simulink model "Robot2R_dyn"  (R2025b)
settings: Solver=VariableStepAuto  StartTime=0.0  StopTime=10.0  RelTol=1e-3  AbsTol=1e-3
undefined symbols (not defined in the file): X, Y, Z
libraries: sm_lib x20, nesl_utility x19, robotcorelib x2, simulink x1
settings Model: Creator=samu0  LastModifiedBy=samuisa
settings SolverCC: AutoScaleAbsTol=off  AlgebraicLoopSolver=TrustRegion  MaxZcPerStep=1.0
settings DebuggingCC: UnconnectedInputMsg=warning  UnconnectedOutputMsg=warning  UnconnectedLineMsg=warning  SymbolicDimsDataTypeCodeGenerationDiagnostic=none
settings ModelReferenceCC: EnableRefExpFcnMdlSchedulingChecks=on
settings SFSimCC: CustomCodeUndefinedFunction=UseInterfaceOnly
settings RTWCC: GPUComputeCapability=3.5  DLArmComputeVersion=19.05
settings SimscapeCC: SimscapeLogType=all  SimscapeLogSimulationStatistics=on  SimscapeLogDataHistory=10000.0

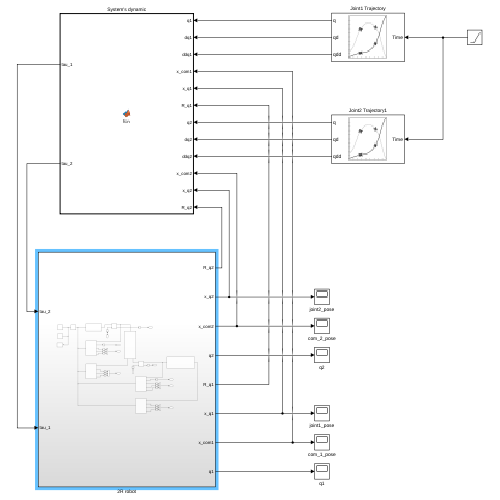
[thumbnail: Simulink's stored preview of the top-level diagram]
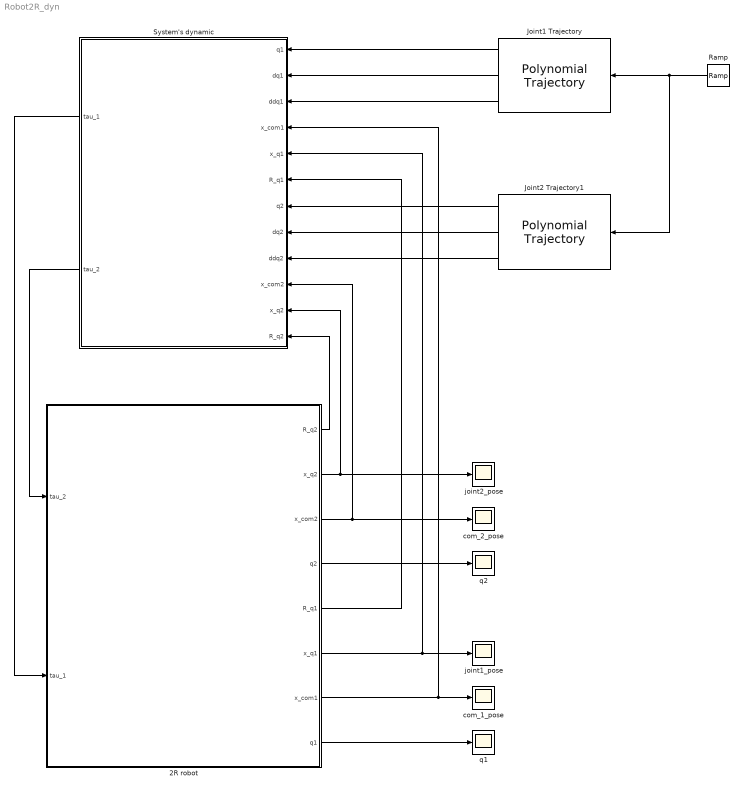
== system Robot2R_dyn ==
  2R robot : Subsystem
  Joint1 Trajectory : robotcorelib/Polynomial Trajectory  WaypointSource=Internal  Waypoints=[ 0, 1.57/2 ]  TimePoints=[ 0, 20 ]  TimeInterval=[ 1, 4 ]  Method=Cubic Polynomial  ParameterSource=Internal  VelocityBoundaryCondition=zeros( 1,2 )  AccelerationBoundaryCondition=zeros( 2, 5 )  SimulateUsing=Interpreted execution
  Joint2 Trajectory1 : robotcorelib/Polynomial Trajectory  WaypointSource=Internal  Waypoints=[ 0, 0 ]  TimePoints=[ 0, 20 ]  TimeInterval=[ 1, 4 ]  Method=Cubic Polynomial  ParameterSource=Internal  VelocityBoundaryCondition=zeros( 1,2 )  AccelerationBoundaryCondition=zeros( 2, 5 )  SimulateUsing=Interpreted execution
  Ramp : simulink/Sources/Ramp  slope=1  start=0  InitialOutput=0
  System's dynamic : MATLAB Function  TreatAsAtomicUnit=on
  com_1_pose : Scope
      settings: ActiveDisplayYMinimum=-1  ActiveDisplayYMaximum=1  DataLoggingVariableName=ScopeData3
  com_2_pose : Scope
      settings: DataLoggingVariableName=ScopeData5
  joint1_pose : Scope
      settings: ActiveDisplayYMinimum=-1  ActiveDisplayYMaximum=1  DataLoggingVariableName=ScopeData2
  joint2_pose : Scope
      settings: DataLoggingVariableName=ScopeData4
  q1 : Scope
  q2 : Scope
  wires:
  System's dynamic/2(tau_2) -> 2R robot/1(tau_2)
  2R robot/7(x_com1) -> com_1_pose/1, System's dynamic/4(x_com1)
  2R robot/3(x_com2) -> com_2_pose/1, System's dynamic/10(x_com2)
  2R robot/8(q1) -> q1/1
  2R robot/4(q2) -> q2/1
  2R robot/2(x_q2) -> joint2_pose/1, System's dynamic/11(x_q2)
  2R robot/6(x_q1) -> joint1_pose/1, System's dynamic/5(x_q1)
  System's dynamic/1(tau_1) -> 2R robot/2(tau_1)
  2R robot/5(R_q1) -> System's dynamic/6(R_q1)
  2R robot/1(R_q2) -> System's dynamic/12(R_q2)
  Joint1 Trajectory/1 -> System's dynamic/1(q1)
  Joint1 Trajectory/2 -> System's dynamic/2(dq1)
  Joint1 Trajectory/3 -> System's dynamic/3(ddq1)
  Joint2 Trajectory1/1 -> System's dynamic/7(q2)
  Joint2 Trajectory1/2 -> System's dynamic/8(dq2)
  Joint2 Trajectory1/3 -> System's dynamic/9(ddq2)
  Ramp/1 -> Joint2 Trajectory1/1, Joint1 Trajectory/1

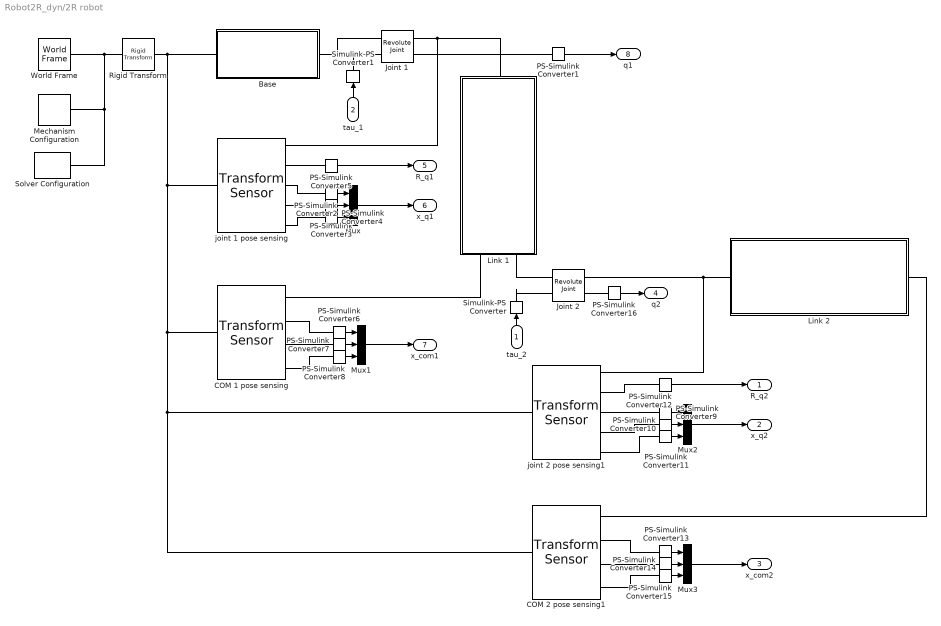
== system Robot2R_dyn/2R robot ==
  tau_2 : Inport
  tau_1 : Inport  Port=2
  Base : Subsystem
  COM 1 pose sensing : sm_lib/Frames and Transforms/Transform Sensor  MeasurementFrame=Base  RotationSequence=XYX  SenseAngle=off  SenseAxis=off  SenseQ=off  SenseR=off  SenseRotationSequence=off  SenseOmegaX=off  SenseOmegaY=off  SenseOmegaZ=off  SenseOmega=off  SenseQDot=off  SenseRDot=off  SenseRotationSequenceDot=off  SenseAlphaX=off  SenseAlphaY=off  SenseAlphaZ=off  SenseAlpha=off  SenseQDDot=off  SenseRDDot=off  SenseX=on  SenseY=on  SenseZ=on  SenseXYZ=off  SenseRad=off  SenseAzim=off  SenseDist=off  SenseInc=off  SenseXDot=off  SenseYDot=off  SenseZDot=off  SenseXYZDot=off  SenseRadDot=off  SenseAzimDot=off  SenseDistDot=off  SenseIncDot=off  SenseXDDot=off  SenseYDDot=off  SenseZDDot=off  SenseXYZDDot=off  SenseRadDDot=off  SenseAzimDDot=off  SenseDistDDot=off  SenseIncDDot=off
  COM 2 pose sensing1 : sm_lib/Frames and Transforms/Transform Sensor  MeasurementFrame=Base  RotationSequence=XYX  SenseAngle=off  SenseAxis=off  SenseQ=off  SenseR=off  SenseRotationSequence=off  SenseOmegaX=off  SenseOmegaY=off  SenseOmegaZ=off  SenseOmega=off  SenseQDot=off  SenseRDot=off  SenseRotationSequenceDot=off  SenseAlphaX=off  SenseAlphaY=off  SenseAlphaZ=off  SenseAlpha=off  SenseQDDot=off  SenseRDDot=off  SenseX=on  SenseY=on  SenseZ=on  SenseXYZ=off  SenseRad=off  SenseAzim=off  SenseDist=off  SenseInc=off  SenseXDot=off  SenseYDot=off  SenseZDot=off  SenseXYZDot=off  SenseRadDot=off  SenseAzimDot=off  SenseDistDot=off  SenseIncDot=off  SenseXDDot=off  SenseYDDot=off  SenseZDDot=off  SenseXYZDDot=off  SenseRadDDot=off  SenseAzimDDot=off  SenseDistDDot=off  SenseIncDDot=off
  Joint 1 : sm_lib/Joints/Revolute Joint  JointMode=Normal  CompositeWrenchDir=FollowerOnBase  CompositeWrenchFrame=BaseFrame  SenseConstraintForce=off  SenseConstraintTorque=off  SenseTotalForce=off  SenseTotalTorque=off  PositionTargetSpecify=off  PositionTargetPriority=High  PositionTargetValue=0  PositionTargetValueUnits=deg  VelocityTargetSpecify=off  VelocityTargetPriority=High  VelocityTargetValue=0  VelocityTargetValueUnits=deg/s  EquilibriumPosition=0  EquilibriumPositionUnits=rad  SpringStiffness=0  SpringStiffnessUnits=N*m/rad  DampingCoefficient=0.002  DampingCoefficientUnits=N*m*s/rad  LowerLimitSpecify=off  LowerLimitBound=-90  LowerLimitBoundUnits=deg  LowerLimitStiffness=1e4  LowerLimitStiffnessUnits=N*m/deg  LowerLimitDamping=10  LowerLimitDampingUnits=N*m/(deg/s)  LowerLimitTransitionRegionWidth=0.1  LowerLimitTransitionRegionWidthUnits=deg  UpperLimitSpecify=off  UpperLimitBound=90  UpperLimitBoundUnits=deg  UpperLimitStiffness=1e4  UpperLimitStiffnessUnits=N*m/deg  UpperLimitDamping=10  UpperLimitDampingUnits=N*m/(deg/s)  UpperLimitTransitionRegionWidth=0.1  UpperLimitTransitionRegionWidthUnits=deg  TorqueActuationMode=InputTorque  MotionActuationMode=ComputedMotion  SensePosition=on  SenseVelocity=off  SenseAcceleration=off  SenseTorqueForce=off  SenseLowerLimitTorqueForce=off  SenseUpperLimitTorqueForce=off
  Joint 2 : sm_lib/Joints/Revolute Joint  JointMode=Normal  CompositeWrenchDir=FollowerOnBase  CompositeWrenchFrame=BaseFrame  SenseConstraintForce=off  SenseConstraintTorque=off  SenseTotalForce=off  SenseTotalTorque=off  PositionTargetSpecify=off  PositionTargetPriority=High  PositionTargetValue=0  PositionTargetValueUnits=deg  VelocityTargetSpecify=off  VelocityTargetPriority=High  VelocityTargetValue=0  VelocityTargetValueUnits=deg/s  EquilibriumPosition=0  EquilibriumPositionUnits=rad  SpringStiffness=0  SpringStiffnessUnits=N*m/rad  DampingCoefficient=0.002  DampingCoefficientUnits=N*m*s/rad  LowerLimitSpecify=off  LowerLimitBound=-90  LowerLimitBoundUnits=deg  LowerLimitStiffness=1e4  LowerLimitStiffnessUnits=N*m/deg  LowerLimitDamping=10  LowerLimitDampingUnits=N*m/(deg/s)  LowerLimitTransitionRegionWidth=0.1  LowerLimitTransitionRegionWidthUnits=deg  UpperLimitSpecify=off  UpperLimitBound=90  UpperLimitBoundUnits=deg  UpperLimitStiffness=1e4  UpperLimitStiffnessUnits=N*m/deg  UpperLimitDamping=10  UpperLimitDampingUnits=N*m/(deg/s)  UpperLimitTransitionRegionWidth=0.1  UpperLimitTransitionRegionWidthUnits=deg  TorqueActuationMode=InputTorque  MotionActuationMode=ComputedMotion  SensePosition=on  SenseVelocity=off  SenseAcceleration=off  SenseTorqueForce=off  SenseLowerLimitTorqueForce=off  SenseUpperLimitTorqueForce=off
  Link 1 : Subsystem
  Link 2 : Subsystem
  Mechanism Configuration : sm_lib/Utilities/Mechanism Configuration  UniformGravity=Constant  GravityVector=[0 0 -9.81]  GravityVectorUnits=m/s^2  LinearizationDelta=0.001  JointModeTransitionNonlinearIterations=2
  Mux{,1..3} (4 alike) : Mux  Inputs=3
  PS-Simulink Converter{1..16} (16 alike) : nesl_utility/PS-Simulink Converter  PhysicalDomain=network_engine_domain  SubClassName=ps_output  LeftPortType=input  RightPortType=output  PseudoPeriodic=off  Frequencies=[]  VectorFormat=inherit  Unit=inherit  AffineConversion=off
  Rigid Transform : sm_lib/Frames and Transforms/Rigid Transform  RotationMethod=AlignedAxes  FollAlignAxisA=+Z  BaseAlignAxisA=-Y  FollAlignAxisB=+X  BaseAlignAxisB=+X  RotationStandardAxis=+Z  RotationAngle=0  RotationAngleUnits=deg  RotationArbitraryAxis=[0 0 1]  RotationSequenceAxes=FollowerAxes  RotationSequence=XYX  RotationSequenceAngles=[0 0 0]  RotationSequenceAnglesUnits=deg  RotationMatrix=[1 0 0;0 1 0;0 0 1]  Quaternion=[1 0 0 0]  TranslationMethod=None  TranslationCartesianOffset=[0 0 0]  TranslationCartesianOffsetUnits=m  TranslationStandardAxis=+Z  TranslationStandardOffset=0  TranslationStandardOffsetUnits=m  TranslationROffset=0  TranslationROffsetUnits=m  TranslationThetaOffset=0  TranslationThetaOffsetUnits=deg  TranslationZOffset=0  TranslationZOffsetUnits=m
  Simulink-PS Converter : nesl_utility/Simulink-PS Converter  PhysicalDomain=network_engine_domain  SubClassName=ps_input  LeftPortType=input  RightPortType=output  PseudoPeriodic=off  Frequencies=[]  NoiseDistribution=none  NoiseParameters=[]  Unit=1  AffineConversion=off  FilteringAndDerivatives=provide  SimscapeFilterOrder=1  InputFilterTimeConstant=0.001  UdotUserProvided=0
  Simulink-PS Converter1 : nesl_utility/Simulink-PS Converter  PhysicalDomain=network_engine_domain  SubClassName=ps_input  LeftPortType=input  RightPortType=output  PseudoPeriodic=off  Frequencies=[]  NoiseDistribution=none  NoiseParameters=[]  Unit=1  AffineConversion=off  FilteringAndDerivatives=provide  SimscapeFilterOrder=1  InputFilterTimeConstant=0.001  UdotUserProvided=0
  Solver Configuration : nesl_utility/Solver Configuration  PhysicalDomain=network_engine_domain  SubClassName=solver  LeftPortType=input  RightPortType=generic  Tones=[]  Harmonics=[]  SimulateNoise=off  Profile=off  UseLocalSampling=off  EnableSwitchedLinearOptims=on  FrequencyDomain=off  UseCCode=off  RelTol=0.001  AbsTol=1e-06  MinStep=1e-09  ToWorkspace=off  RevertToSquareIcSolve=off  NumHomotopyIterations=100  PhasorMode=off  PhasorModeNumHarmonics=1  ConsistencySolver=NEWTON_XTOL_AFTER_FTOL  IndexReductionMethod=DerivativeReplacement  DoDC=off  ResidualTolerance=1e-09  ConsistencyTolSource=GLOBAL  ConsistencyAbsTol=0.001  ConsistencyRelTol=0.001  ConsistencyTolFactor=0.001  UseLocalSolver=off  LocalSolverChoice=NE_BACKWARD_EULER_ADVANCER  ResolveIndetEquations=on  FunctionEvalNumThread=1  LocalSolverSampleTime=0.001  DoFixedCost=off  MaxNonlinIter=3  MaxModeIter=2  ComputeImpulses=off  ImpulseIterations=2  LinearAlgebra=auto  LinearAlgebraNumThread=0  EquationFormulation=NE_TIME_EF  DelaysMemoryBudget=1024  AutomaticFiltering=on  FilteringTimeConstant=0.001  PartitionStorageMethod=AS_NEEDED  PartitionMemoryBudget=1024  PartitionMethod=ROBUST  MultibodyUseLocalSolver=off  MultibodyLocalSolverChoice=ODE1  MultibodyLocalSolverSampleTime=0.001
  World Frame : sm_lib/Frames and Transforms/World Frame
  joint 1 pose sensing : sm_lib/Frames and Transforms/Transform Sensor  MeasurementFrame=Base  RotationSequence=XYX  SenseAngle=off  SenseAxis=off  SenseQ=off  SenseR=on  SenseRotationSequence=off  SenseOmegaX=off  SenseOmegaY=off  SenseOmegaZ=off  SenseOmega=off  SenseQDot=off  SenseRDot=off  SenseRotationSequenceDot=off  SenseAlphaX=off  SenseAlphaY=off  SenseAlphaZ=off  SenseAlpha=off  SenseQDDot=off  SenseRDDot=off  SenseX=on  SenseY=on  SenseZ=on  SenseXYZ=off  SenseRad=off  SenseAzim=off  SenseDist=off  SenseInc=off  SenseXDot=off  SenseYDot=off  SenseZDot=off  SenseXYZDot=off  SenseRadDot=off  SenseAzimDot=off  SenseDistDot=off  SenseIncDot=off  SenseXDDot=off  SenseYDDot=off  SenseZDDot=off  SenseXYZDDot=off  SenseRadDDot=off  SenseAzimDDot=off  SenseDistDDot=off  SenseIncDDot=off
  joint 2 pose sensing1 : sm_lib/Frames and Transforms/Transform Sensor  MeasurementFrame=Base  RotationSequence=XYX  SenseAngle=off  SenseAxis=off  SenseQ=off  SenseR=on  SenseRotationSequence=off  SenseOmegaX=off  SenseOmegaY=off  SenseOmegaZ=off  SenseOmega=off  SenseQDot=off  SenseRDot=off  SenseRotationSequenceDot=off  SenseAlphaX=off  SenseAlphaY=off  SenseAlphaZ=off  SenseAlpha=off  SenseQDDot=off  SenseRDDot=off  SenseX=on  SenseY=on  SenseZ=on  SenseXYZ=off  SenseRad=off  SenseAzim=off  SenseDist=off  SenseInc=off  SenseXDot=off  SenseYDot=off  SenseZDot=off  SenseXYZDot=off  SenseRadDot=off  SenseAzimDot=off  SenseDistDot=off  SenseIncDot=off  SenseXDDot=off  SenseYDDot=off  SenseZDDot=off  SenseXYZDDot=off  SenseRadDDot=off  SenseAzimDDot=off  SenseDistDDot=off  SenseIncDDot=off
  R_q2 : Outport
  x_q2 : Outport  Port=2
  x_com2 : Outport  Port=3
  q2 : Outport  Port=4
  R_q1 : Outport  Port=5
  x_q1 : Outport  Port=6
  x_com1 : Outport  Port=7
  q1 : Outport  Port=8
  wires:
  PS-Simulink Converter13/1 -> Mux3/1
  PS-Simulink Converter15/1 -> Mux3/3
  Mux3/1 -> x_com2/1
  PS-Simulink Converter5/1 -> R_q1/1
  Mux1/1 -> x_com1/1
  PS-Simulink Converter8/1 -> Mux1/3
  PS-Simulink Converter12/1 -> R_q2/1
  Mux2/1 -> x_q2/1
  PS-Simulink Converter4/1 -> Mux/3
  PS-Simulink Converter3/1 -> Mux/2
  PS-Simulink Converter14/1 -> Mux3/2
  PS-Simulink Converter10/1 -> Mux2/2
  PS-Simulink Converter9/1 -> Mux2/1
  Mux/1 -> x_q1/1
  PS-Simulink Converter6/1 -> Mux1/1
  PS-Simulink Converter7/1 -> Mux1/2
  PS-Simulink Converter1/1 -> q1/1
  PS-Simulink Converter11/1 -> Mux2/3
  PS-Simulink Converter2/1 -> Mux/1
  PS-Simulink Converter16/1 -> q2/1
  tau_2/1 -> Simulink-PS Converter/1
  tau_1/1 -> Simulink-PS Converter1/1
  connections:
  COM 1 pose sensing/RConn4 -- PS-Simulink Converter8/LConn1
  joint 2 pose sensing1/RConn1 -- Joint 2/RConn1 -- Link 2/LConn1
  Solver Configuration/RConn1 -- Mechanism Configuration/RConn1 -- World Frame/RConn1 -- Rigid Transform/LConn1
  Base/RConn1 -- Joint 1/LConn1
  PS-Simulink Converter12/LConn1 -- joint 2 pose sensing1/RConn2
  PS-Simulink Converter5/LConn1 -- joint 1 pose sensing/RConn2
  joint 2 pose sensing1/RConn5 -- PS-Simulink Converter11/LConn1
  COM 1 pose sensing/RConn3 -- PS-Simulink Converter7/LConn1
  joint 1 pose sensing/RConn1 -- Link 1/LConn1 -- Joint 1/RConn1
  COM 2 pose sensing1/RConn3 -- PS-Simulink Converter14/LConn1
  joint 1 pose sensing/RConn3 -- PS-Simulink Converter2/LConn1
  COM 2 pose sensing1/RConn2 -- PS-Simulink Converter13/LConn1
  joint 1 pose sensing/RConn4 -- PS-Simulink Converter3/LConn1
  COM 1 pose sensing/RConn2 -- PS-Simulink Converter6/LConn1
  COM 2 pose sensing1/RConn4 -- PS-Simulink Converter15/LConn1
  PS-Simulink Converter1/LConn1 -- Joint 1/RConn2
  joint 2 pose sensing1/RConn3 -- PS-Simulink Converter9/LConn1
  joint 1 pose sensing/RConn5 -- PS-Simulink Converter4/LConn1
  Link 2/RConn1 -- COM 2 pose sensing1/RConn1
  Joint 2/LConn1 -- Link 1/RConn2
  joint 2 pose sensing1/RConn4 -- PS-Simulink Converter10/LConn1
  COM 1 pose sensing/RConn1 -- Link 1/RConn1
  PS-Simulink Converter16/LConn1 -- Joint 2/RConn2
  Simulink-PS Converter/RConn1 -- Joint 2/LConn2
  Base/LConn1 -- joint 1 pose sensing/LConn1 -- COM 1 pose sensing/LConn1 -- joint 2 pose sensing1/LConn1 -- COM 2 pose sensing1/LConn1 -- Rigid Transform/RConn1
  Simulink-PS Converter1/RConn1 -- Joint 1/LConn2

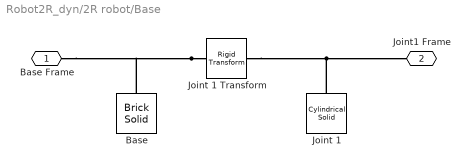
== system Robot2R_dyn/2R robot/Base ==
  Base : sm_lib/Body Elements/Brick Solid  BrickDimensions=[5 5 0.5]  BrickDimensionsUnits=m  ExportEntireGeometry=off  InertiaType=PointMass  BasedOnType=Density  Density=1000  DensityUnits=kg/m^3  Mass=0  MassUnits=kg  CenterOfMass=[0 0 0]  CenterOfMassUnits=m  MomentsOfInertia=[1 1 1]  MomentsOfInertiaUnits=kg*m^2  ProductsOfInertia=[0 0 0]  ProductsOfInertiaUnits=kg*m^2  GraphicType=FromGeometry  MarkerShape=Sphere  MarkerSize=10  GraphicVisPropType=SimpleVisualProperties  GraphicDiffuseColor=[1 1 0]  GraphicOpacity=1  GraphicSpecularColor=[0.5 0.5 0.5 1.0]  GraphicAmbientColor=[0.15 0.15 0.15 1.0]  GraphicEmissiveColor=[0.0 0.0 0.0 1.0]  GraphicShininess=75  DoExposeReferenceFrame=on  SerializedFrames=<Frames/>
  Joint 1 : sm_lib/Body Elements/Cylindrical Solid  CylinderRadius=0.5  CylinderRadiusUnits=m  CylinderLength=0.6  CylinderLengthUnits=m  ExportEntireGeometry=off  InertiaType=PointMass  BasedOnType=Density  Density=1000  DensityUnits=kg/m^3  Mass=0  MassUnits=kg  CenterOfMass=[0 0 0]  CenterOfMassUnits=m  MomentsOfInertia=[1 1 1]  MomentsOfInertiaUnits=kg*m^2  ProductsOfInertia=[0 0 0]  ProductsOfInertiaUnits=kg*m^2  GraphicType=FromGeometry  MarkerShape=Sphere  MarkerSize=10  GraphicVisPropType=SimpleVisualProperties  GraphicDiffuseColor=[1 0 1]  GraphicOpacity=1  GraphicSpecularColor=[0.5 0.5 0.5 1.0]  GraphicAmbientColor=[0.15 0.15 0.15 1.0]  GraphicEmissiveColor=[0.0 0.0 0.0 1.0]  GraphicShininess=75  DoExposeReferenceFrame=on  SerializedFrames=<Frames/>
  Joint 1 Transform : sm_lib/Frames and Transforms/Rigid Transform  RotationMethod=AlignedAxes  FollAlignAxisA=+Y  BaseAlignAxisA=+Y  FollAlignAxisB=+X  BaseAlignAxisB=+X  RotationStandardAxis=+Z  RotationAngle=0  RotationAngleUnits=deg  RotationArbitraryAxis=[0 0 1]  RotationSequenceAxes=FollowerAxes  RotationSequence=XYX  RotationSequenceAngles=[0 0 0]  RotationSequenceAnglesUnits=deg  RotationMatrix=[1 0 0;0 1 0;0 0 1]  Quaternion=[1 0 0 0]  TranslationMethod=StandardAxis  TranslationCartesianOffset=[0 0 0]  TranslationCartesianOffsetUnits=m  TranslationStandardAxis=+Z  TranslationStandardOffset=0.5  TranslationStandardOffsetUnits=m  TranslationROffset=0  TranslationROffsetUnits=m  TranslationThetaOffset=0  TranslationThetaOffsetUnits=deg  TranslationZOffset=0  TranslationZOffsetUnits=m
  Base Frame : PMIOPort  Side=Left
  Joint1 Frame : PMIOPort  Port=2  Side=Right
  connections:
  Joint 1 Transform/LConn1 -- Base Frame/RConn1 -- Base/RConn1
  Joint 1 Transform/RConn1 -- Joint1 Frame/RConn1 -- Joint 1/RConn1

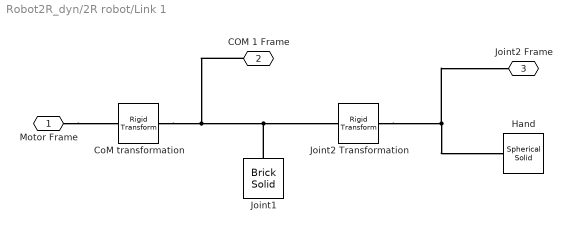
== system Robot2R_dyn/2R robot/Link 1 ==
  CoM transformation : sm_lib/Frames and Transforms/Rigid Transform  RotationMethod=None  FollAlignAxisA=+X  BaseAlignAxisA=+Y  FollAlignAxisB=+Y  BaseAlignAxisB=+Z  RotationStandardAxis=+Z  RotationAngle=0  RotationAngleUnits=deg  RotationArbitraryAxis=[0 0 1]  RotationSequenceAxes=FollowerAxes  RotationSequence=XYX  RotationSequenceAngles=[0 0 0]  RotationSequenceAnglesUnits=deg  RotationMatrix=[1 0 0;0 1 0;0 0 1]  Quaternion=[1 0 0 0]  TranslationMethod=StandardAxis  TranslationCartesianOffset=[0 0 0]  TranslationCartesianOffsetUnits=m  TranslationStandardAxis=+X  TranslationStandardOffset=2.5  TranslationStandardOffsetUnits=m  TranslationROffset=0  TranslationROffsetUnits=m  TranslationThetaOffset=0  TranslationThetaOffsetUnits=deg  TranslationZOffset=0  TranslationZOffsetUnits=m
  Hand : sm_lib/Body Elements/Spherical Solid  SphereRadius=0.5  SphereRadiusUnits=m  ExportEntireGeometry=off  InertiaType=PointMass  BasedOnType=Density  Density=1000  DensityUnits=kg/m^3  Mass=0  MassUnits=kg  CenterOfMass=[0 0 0]  CenterOfMassUnits=m  MomentsOfInertia=[1 1 1]  MomentsOfInertiaUnits=kg*m^2  ProductsOfInertia=[0 0 0]  ProductsOfInertiaUnits=kg*m^2  GraphicType=FromGeometry  MarkerShape=Sphere  MarkerSize=10  GraphicVisPropType=SimpleVisualProperties  GraphicDiffuseColor=[0 0 1]  GraphicOpacity=1  GraphicSpecularColor=[0.5 0.5 0.5 1.0]  GraphicAmbientColor=[0.15 0.15 0.15 1.0]  GraphicEmissiveColor=[0.0 0.0 0.0 1.0]  GraphicShininess=75  DoExposeReferenceFrame=on  SerializedFrames=<Frames/>
  Joint1 : sm_lib/Body Elements/Brick Solid  BrickDimensions=[5 0.5 0.5]  BrickDimensionsUnits=m  ExportEntireGeometry=off  InertiaType=PointMass  BasedOnType=Mass  Density=1000  DensityUnits=kg/m^3  Mass=1  MassUnits=kg  CenterOfMass=[0 0 0]  CenterOfMassUnits=m  MomentsOfInertia=[1 1 1]  MomentsOfInertiaUnits=kg*m^2  ProductsOfInertia=[0 0 0]  ProductsOfInertiaUnits=kg*m^2  GraphicType=FromGeometry  MarkerShape=Sphere  MarkerSize=10  GraphicVisPropType=SimpleVisualProperties  GraphicDiffuseColor=[1 0 0]  GraphicOpacity=1  GraphicSpecularColor=[0.5 0.5 0.5 1.0]  GraphicAmbientColor=[0.15 0.15 0.15 1.0]  GraphicEmissiveColor=[0.0 0.0 0.0 1.0]  GraphicShininess=75  DoExposeReferenceFrame=on  SerializedFrames=<Frames/>
  Joint2 Transformation : sm_lib/Frames and Transforms/Rigid Transform  RotationMethod=None  FollAlignAxisA=+X  BaseAlignAxisA=+Y  FollAlignAxisB=+Y  BaseAlignAxisB=+Z  RotationStandardAxis=+Z  RotationAngle=0  RotationAngleUnits=deg  RotationArbitraryAxis=[0 0 1]  RotationSequenceAxes=FollowerAxes  RotationSequence=XYX  RotationSequenceAngles=[0 0 0]  RotationSequenceAnglesUnits=deg  RotationMatrix=[1 0 0;0 1 0;0 0 1]  Quaternion=[1 0 0 0]  TranslationMethod=StandardAxis  TranslationCartesianOffset=[0 0 0]  TranslationCartesianOffsetUnits=m  TranslationStandardAxis=+X  TranslationStandardOffset=2.5  TranslationStandardOffsetUnits=m  TranslationROffset=0  TranslationROffsetUnits=m  TranslationThetaOffset=0  TranslationThetaOffsetUnits=deg  TranslationZOffset=0  TranslationZOffsetUnits=m
  Motor Frame : PMIOPort  Side=Left
  COM 1 Frame : PMIOPort  Port=2  Side=Right
  Joint2 Frame : PMIOPort  Port=3  Side=Right
  connections:
  Joint2 Transformation/RConn1 -- Joint2 Frame/RConn1 -- Hand/RConn1
  CoM transformation/RConn1 -- COM 1 Frame/RConn1 -- Joint1/RConn1 -- Joint2 Transformation/LConn1
  Motor Frame/RConn1 -- CoM transformation/LConn1

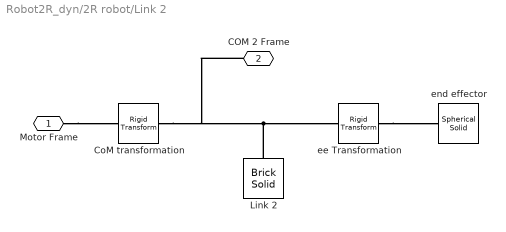
== system Robot2R_dyn/2R robot/Link 2 ==
  CoM transformation : sm_lib/Frames and Transforms/Rigid Transform  RotationMethod=None  FollAlignAxisA=+X  BaseAlignAxisA=+Y  FollAlignAxisB=+Y  BaseAlignAxisB=+Z  RotationStandardAxis=+Z  RotationAngle=0  RotationAngleUnits=deg  RotationArbitraryAxis=[0 0 1]  RotationSequenceAxes=FollowerAxes  RotationSequence=XYX  RotationSequenceAngles=[0 0 0]  RotationSequenceAnglesUnits=deg  RotationMatrix=[1 0 0;0 1 0;0 0 1]  Quaternion=[1 0 0 0]  TranslationMethod=StandardAxis  TranslationCartesianOffset=[0 0 0]  TranslationCartesianOffsetUnits=m  TranslationStandardAxis=+X  TranslationStandardOffset=2.5  TranslationStandardOffsetUnits=m  TranslationROffset=0  TranslationROffsetUnits=m  TranslationThetaOffset=0  TranslationThetaOffsetUnits=deg  TranslationZOffset=0  TranslationZOffsetUnits=m
  Link 2 : sm_lib/Body Elements/Brick Solid  BrickDimensions=[5 0.5 0.5]  BrickDimensionsUnits=m  ExportEntireGeometry=off  InertiaType=CalculateFromGeometry  BasedOnType=Mass  Density=1000  DensityUnits=kg/m^3  Mass=1  MassUnits=kg  CenterOfMass=[0 0 0]  CenterOfMassUnits=m  MomentsOfInertia=[1 1 1]  MomentsOfInertiaUnits=kg*m^2  ProductsOfInertia=[0 0 0]  ProductsOfInertiaUnits=kg*m^2  GraphicType=FromGeometry  MarkerShape=Sphere  MarkerSize=10  GraphicVisPropType=SimpleVisualProperties  GraphicDiffuseColor=[0 1 0]  GraphicOpacity=1  GraphicSpecularColor=[0.5 0.5 0.5 1.0]  GraphicAmbientColor=[0.15 0.15 0.15 1.0]  GraphicEmissiveColor=[0.0 0.0 0.0 1.0]  GraphicShininess=75  DoExposeReferenceFrame=on  SerializedFrames=<Frames/>
  ee Transformation : sm_lib/Frames and Transforms/Rigid Transform  RotationMethod=None  FollAlignAxisA=+X  BaseAlignAxisA=+Y  FollAlignAxisB=+Y  BaseAlignAxisB=+Z  RotationStandardAxis=+Z  RotationAngle=0  RotationAngleUnits=deg  RotationArbitraryAxis=[0 0 1]  RotationSequenceAxes=FollowerAxes  RotationSequence=XYX  RotationSequenceAngles=[0 0 0]  RotationSequenceAnglesUnits=deg  RotationMatrix=[1 0 0;0 1 0;0 0 1]  Quaternion=[1 0 0 0]  TranslationMethod=StandardAxis  TranslationCartesianOffset=[0 0 0]  TranslationCartesianOffsetUnits=m  TranslationStandardAxis=+X  TranslationStandardOffset=2.5  TranslationStandardOffsetUnits=m  TranslationROffset=0  TranslationROffsetUnits=m  TranslationThetaOffset=0  TranslationThetaOffsetUnits=deg  TranslationZOffset=0  TranslationZOffsetUnits=m
  end effector : sm_lib/Body Elements/Spherical Solid  SphereRadius=0.5  SphereRadiusUnits=m  ExportEntireGeometry=off  InertiaType=PointMass  BasedOnType=Density  Density=1000  DensityUnits=kg/m^3  Mass=0  MassUnits=kg  CenterOfMass=[0 0 0]  CenterOfMassUnits=m  MomentsOfInertia=[1 1 1]  MomentsOfInertiaUnits=kg*m^2  ProductsOfInertia=[0 0 0]  ProductsOfInertiaUnits=kg*m^2  GraphicType=FromGeometry  MarkerShape=Sphere  MarkerSize=10  GraphicVisPropType=SimpleVisualProperties  GraphicDiffuseColor=[0 0 1]  GraphicOpacity=1  GraphicSpecularColor=[0.5 0.5 0.5 1.0]  GraphicAmbientColor=[0.15 0.15 0.15 1.0]  GraphicEmissiveColor=[0.0 0.0 0.0 1.0]  GraphicShininess=75  DoExposeReferenceFrame=on  SerializedFrames=<Frames/>
  Motor Frame : PMIOPort  Side=Left
  COM 2 Frame : PMIOPort  Port=2  Side=Right
  connections:
  ee Transformation/RConn1 -- end effector/RConn1
  Link 2/RConn1 -- ee Transformation/LConn1 -- CoM transformation/RConn1 -- COM 2 Frame/RConn1
  Motor Frame/RConn1 -- CoM transformation/LConn1

== matlab function Robot2R_dyn/System's dynamic ==
  data: q1 input; dq1 input; ddq1 input; tau_1 output; x_com1 input; x_q1 input; R_q1 input; tau_2 output; q2 input; dq2 input; ddq2 input; x_com2 input; x_q2 input; R_q2 input
function [tau_1, tau_2] = fcn(q1, dq1, ddq1, x_com1, x_q1, R_q1, q2, dq2, ddq2, x_com2, x_q2, R_q2)
    %% DATA ORGANIZATION

    q = [q1; q2]; dq = [dq1; dq2]; ddq = [ddq1; ddq2];
    m = [1, 1];
    g_mag = 9.81;
    vdot_0 = [0; g_mag; 0]; % Fictitious gravity (pushes the base upwards)
    
    % Relative Rotation Matrices
    R_12 = R_q1' * R_q2;
    R_list = {R_q1, R_12}; % R_list{1} = Rot Base->1, R_list{2} = Rot 1->2
    
    % Center of mass position vectors (expressed in local frames)
    Pc = {R_q1' * (x_com1 - x_q1), R_q2' * (x_com2 - x_q2)};
    
    % Joint position vectors (P{i} = from joint i-1 to joint i, in frame i-1)
    P  = {[0; 0; 0.5], [5; 0; 0]}; 
    
    % Inertias
    I = {diag([0, 1/12*m(1)*(5)^2, 1/12*m(1)*(5)^2]), ...
         diag([0, 1/12*m(2)*(5)^2, 1/12*m(2)*(5)^2])};
    
    % Kinematic variables initialization
    w = zeros(3, 3);
    wd = zeros(3, 3);
    vd = zeros(3, 3);
    
    % <--- FIX 1: APPLY GRAVITY TO THE BASE --->
    vd(:, 1) = vdot_0; 
    
    vdc = zeros(3, 2);
    F = zeros(3, 2);
    N = zeros(3, 2);
    z0 = [0; 0; 1];
    num_joint = 2;
    
    %% FORWARD RECURSION
    for i = 1:num_joint
        idx = i + 1; 
        prev = i;    
        
        Ri = R_list{i}'; % Transpose to pass from the previous frame to the local one
        
        w(:, idx) = Ri * w(:, prev) + dq(i) * z0;
        
        wd(:, idx) = Ri * wd(:, prev) + ...
                     cross(Ri * w(:, prev), dq(i) * z0) + ddq(i) * z0;
        
        vd(:, idx) = Ri * (vd(:, prev) + cross(wd(:, prev), P{i}) + ...
                     cross(w(:, prev), cross(w(:, prev), P{i})));
        
        vdc(:, i) = vd(:, idx) + cross(wd(:, idx), Pc{i}) + ...
                    cross(w(:, idx), cross(w(:, idx), Pc{i}));
        
        F(:, i) = m(i) * vdc(:, i);
        N(:, i) = I{i} * wd(:, idx) + cross(w(:, idx), I{i} * w(:, idx));
    end
    
    %% BACKWARD RECURSION
    f_next = [0;0;0]; 
    n_next = [0;0;0]; 
    tau = zeros(2, 1);
    
    for i = num_joint:-1:1
        % <--- FIX 2 & 3: CORRECT ROTATIONS AND LEVER ARMS --->
        if i == 2
            R_next = eye(3);       % No rotation after the EE (End-Effector)
            P_next = [5; 0; 0];  % Distance Joint2 -> End Effector (link 2 length)
        else
            R_next = R_list{2};    % R_1^2 matrix to rotate forces from Link 2 to Link 1
            P_next = P{2};         % Distance Joint1 -> Joint2
        end
        
        % Rotate the subsequent force into the current frame before adding!
        f_curr = R_next * f_next + F(:, i);
        
        n_curr = N(:, i) + R_next * n_next + ...
                 cross(Pc{i}, F(:, i)) + ...
                 cross(P_next, R_next * f_next); % The correct lever arm with the rotated force
        
        % Torque extraction
        tau(i) = n_curr' * z0;
        
        f_next = f_curr;
        n_next = n_curr;
    end
    
    tau_1 = tau(1);
    tau_2 = tau(2);
end
